simulink model "Solar_track_Lead_Lag"  (R2026b)
settings: Solver=FixedStepAuto  StopTime=60  FixedStep=0.01
InitFcn:
  | Lead_Lag_Controller;
  | Laplace_Simplified;
values from neighbouring files (symbols this model uses):
  den_dist = [1 -3.71131896899 5.17245520139 -3.20991964144 0.74878351206]    [linsys1.mat]
  denCz = [1 -1.74081722068 0.740817479864]    [linsys1.mat]
  denGpos_z = [1 -1.98796767638 0.987967676384]    [linsys1.mat]
  J = J_r + (J_p/N^2)    (= 0.0035)    [Ches_workspace.m]    (also in linsys1.mat = 0.0396; params.m = 0.0396)
  K_a = 0.2    [Ches_workspace.m]    (also in linsys1.mat; params.m)
  K_b = 0.009549    [Ches_workspace.m]    (also in linsys1.mat; params.m)
  K_f = 0.047746    [Ches_workspace.m]    (also in linsys1.mat; params.m)
  K_p = 4    [Ches_workspace.m]    (also in linsys1.mat; params.m)
  K_p2 = 25    [linsys1.mat]    (also in params.m)
  K_s = h*(2/1.8)    (= 1.66666666667)    [Ches_workspace.m]    (also in linsys1.mat = 0.277777777778; params.m = 0.277777777778)
  N = 20    [Ches_workspace.m]    (also in linsys1.mat; params.m)
  num_dist = [0 3.14386705394e-06 -2.34169109534e-06 -3.12182707139e-06 2.31965273917e-06]    [linsys1.mat]
  numCz = [500 -985.172769274 485.174246924]    [linsys1.mat]
  numGpos_z = [0 5.0301872863e-06 5.00993089871e-06]    [linsys1.mat]
  R_m = 10    [Ches_workspace.m]    (also in linsys1.mat; params.m)
undefined symbols (not defined in the file or in its folder): dspblkCoreblockFVToolHelper, gcbh
settings Model: Creator=milan  LastModifiedBy=milan

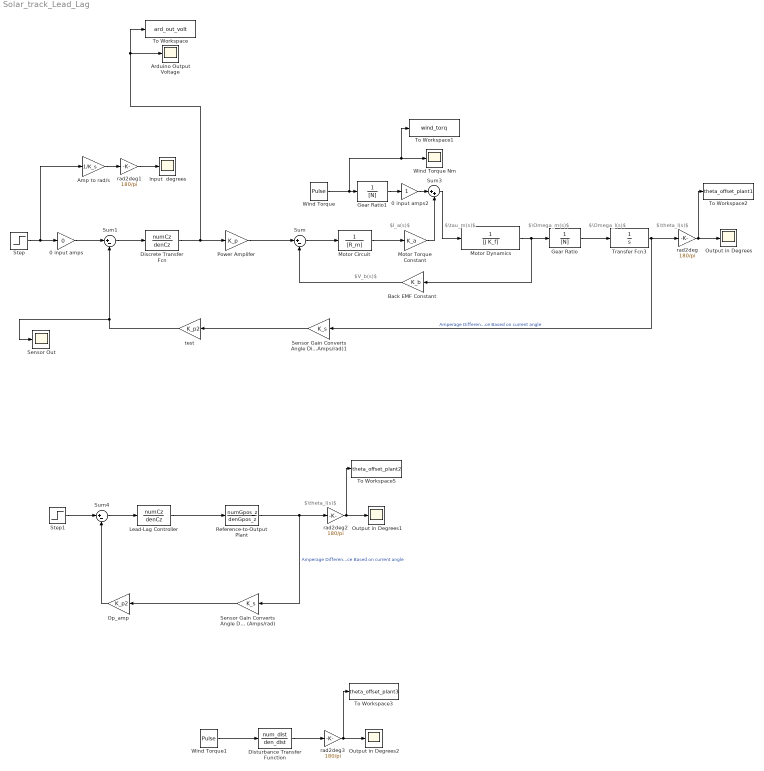
== system Solar_track_Lead_Lag ==
  note: $V_b(s)$
  note: $I_a(s)$
  note: $\tau_m(s)$
  note: $\Omega_m(s)$
  note: $\Omega_l(s)$
  note: $\theta_l(s)$
  note: $\theta_l(s)$
  0 input amps : Gain  Gain=0
  0 input amps2 : Gain
  Amp to rad/s : Gain  Gain=1/K_s
  Arduino Output Voltage : Scope
      settings: ActiveDisplayYMinimum=-110.729181028056  ActiveDisplayYMaximum=93.4022833423949  DataLoggingVariableName=ScopeData3
  Back EMF Constant : Gain  Gain=K_b
  Discrete Transfer Fcn : DiscreteTransferFcn  LoadFcn=dspblkCoreblockFVToolHelper(gcbh,'load');  Numerator=numCz  Denominator=denCz
      settings: CopyFcn=dspblkCoreblockFVToolHelper(gcbh,'copy');  DeleteFcn=dspblkCoreblockFVToolHelper(gcbh,'close');  ModelCloseFcn=dspblkCoreblockFVToolHelper(gcbh,'close');  PreSaveFcn=dspblkCoreblockFVToolHelper(gcbh,'presave');  PostSaveFcn=dspblkCoreblockFVToolHelper(gcbh,'postsave');  CloseFcn=dspblkCoreblockFVToolHelper(gcbh,'close');
  Disturbance Transfer Function : DiscreteTransferFcn  Numerator=num_dist  Denominator=den_dist
  Gear Ratio : TransferFcn  Denominator=[N]
  Gear Ratio1 : TransferFcn  Denominator=[N]
  Input  degrees : Scope
      settings: ActiveDisplayYMinimum=-14.30826241958318  ActiveDisplayYMaximum=86.208767418503754
  Lead-Lag Controller : DiscreteTransferFcn  LoadFcn=dspblkCoreblockFVToolHelper(gcbh,'load');  Numerator=numCz  Denominator=denCz
      settings: CopyFcn=dspblkCoreblockFVToolHelper(gcbh,'copy');  DeleteFcn=dspblkCoreblockFVToolHelper(gcbh,'close');  ModelCloseFcn=dspblkCoreblockFVToolHelper(gcbh,'close');  PreSaveFcn=dspblkCoreblockFVToolHelper(gcbh,'presave');  PostSaveFcn=dspblkCoreblockFVToolHelper(gcbh,'postsave');  CloseFcn=dspblkCoreblockFVToolHelper(gcbh,'close');
  Motor Circuit : TransferFcn  Denominator=[R_m]
  Motor Dynamics : TransferFcn  Denominator=[J K_f]
  Motor Torque Constant : Gain  Gain=K_a
  Op_amp : Gain  Gain=K_p2
  Output in Degrees : Scope
      settings: ActiveDisplayYMinimum=-1.2014189631595029  ActiveDisplayYMaximum=10.812770668435528
  Output in Degrees1 : Scope
      settings: ActiveDisplayYMinimum=-1.2014185941625415  ActiveDisplayYMaximum=10.812767347462875  DataLoggingVariableName=ScopeData6
  Output in Degrees2 : Scope
      settings: ActiveDisplayYMinimum=-3.5279281348796792  ActiveDisplayYMaximum=15.46041956703375  DataLoggingVariableName=ScopeData4
  Power Amplifer : Gain  Gain=K_p
  Reference-to-Output Plant : DiscreteTransferFcn  Numerator=numGpos_z  Denominator=denGpos_z
  Sensor Gain Converts Angle Difference into amp difference (Amps/rad) : Gain  Gain=K_s
  Sensor Gain Converts Angle Difference into amp difference (Amps/rad)1 : Gain  Gain=K_s
  Sensor Out : Scope
      settings: ActiveDisplayYMinimum=-837.568627409983  ActiveDisplayYMaximum=365.83860161490566  DataLoggingVariableName=ScopeData11
  Step : Step  Time=0.01  SampleTime=0.01
  Step1 : Step  Time=0.01  SampleTime=0.01
  Sum : Sum  Inputs=|+-
  Sum1 : Sum  Inputs=|+-
  Sum3 : Sum  Inputs=|++
  Sum4 : Sum  Inputs=|+-
  To Workspace : ToWorkspace  VariableName=ard_out_volt  SaveFormat=Timeseries  SampleTime=-1
  To Workspace1 : ToWorkspace  VariableName=wind_torq  SaveFormat=Timeseries  SampleTime=-1
  To Workspace2 : ToWorkspace  VariableName=theta_offset_plant1  SaveFormat=Timeseries  SampleTime=-1
  To Workspace3 : ToWorkspace  VariableName=theta_offset_plant3  SaveFormat=Timeseries  SampleTime=-1
  To Workspace5 : ToWorkspace  VariableName=theta_offset_plant2  SaveFormat=Timeseries  SampleTime=-1
  Transfer Fcn3 : TransferFcn  Denominator=[1 0]
  Wind Torque : DiscretePulseGenerator  PulseType=Time based  Amplitude=100  Period=500
  Wind Torque Nm : Scope
      settings: ActiveDisplayYMinimum=-0.12499999999999997  ActiveDisplayYMaximum=1.125  DataLoggingVariableName=ScopeData2
  Wind Torque1 : DiscretePulseGenerator  PulseType=Time based  Amplitude=100  Period=500
  rad2deg{,1..3} (4 alike) : Gain  Gain=180/pi
  test : Gain  Gain=K_p2
  wires:
  Motor Circuit/1 -> Motor Torque Constant/1
  Motor Torque Constant/1 -> Sum3/2
  Motor Dynamics/1 -> Gear Ratio/1, Back EMF Constant/1
  Gear Ratio/1 -> Transfer Fcn3/1
  Transfer Fcn3/1 -> Sensor Gain Converts Angle Difference into amp difference (Amps/rad)1/1, rad2deg/1  "Amperage Difference Based on current angle"
  Back EMF Constant/1 -> Sum/2
  Sum/1 -> Motor Circuit/1
  rad2deg/1 -> To Workspace2/1, Output in Degrees/1
  Step/1 -> 0 input amps/1, Amp to rad/s/1
  Amp to rad/s/1 -> rad2deg1/1
  rad2deg1/1 -> Input  degrees/1
  0 input amps/1 -> Sum1/1
  Sum3/1 -> Motor Dynamics/1
  Wind Torque/1 -> To Workspace1/1, Wind Torque Nm/1, Gear Ratio1/1
  Gear Ratio1/1 -> 0 input amps2/1
  Sum1/1 -> Discrete Transfer Fcn/1
  0 input amps2/1 -> Sum3/1
  Discrete Transfer Fcn/1 -> Power Amplifer/1, To Workspace/1, Arduino Output Voltage/1
  Power Amplifer/1 -> Sum/1
  Sensor Gain Converts Angle Difference into amp difference (Amps/rad)1/1 -> test/1
  Reference-to-Output Plant/1 -> Sensor Gain Converts Angle Difference into amp difference (Amps/rad)/1, rad2deg2/1  "Amperage Difference Based on current angle"
  Step1/1 -> Sum4/1
  Sensor Gain Converts Angle Difference into amp difference (Amps/rad)/1 -> Op_amp/1
  Lead-Lag Controller/1 -> Reference-to-Output Plant/1
  Sum4/1 -> Lead-Lag Controller/1
  rad2deg2/1 -> To Workspace5/1, Output in Degrees1/1
  test/1 -> Sensor Out/1, Sum1/2
  Op_amp/1 -> Sum4/2
  rad2deg3/1 -> To Workspace3/1, Output in Degrees2/1
  Wind Torque1/1 -> Disturbance Transfer Function/1
  Disturbance Transfer Function/1 -> rad2deg3/1
